simulink model "grid_inv_test_battery"  (R2023a)
settings: Solver=FixedStepDiscrete  StartTime=0.0  StopTime=0.6  FixedStep=5e-6  RelTol=1e-3
libraries: spsSeriesRLCBranchLib x8, slpidlib x4, spsVoltageMeasurementLib x4, spsDiodeLib x3, spsCurrentMeasurementLib x2, spsUniversalBridgeLib x2, spsPVArrayLib x2, spsPWMGenerator2LevelLib x2, spsabctodq0Lib x2, spsDCVoltageSourceLib x1, spsThreePhaseFaultLib x1, spsIGBTLib x1
settings Model: Creator=Umer  LastModifiedBy=Umer

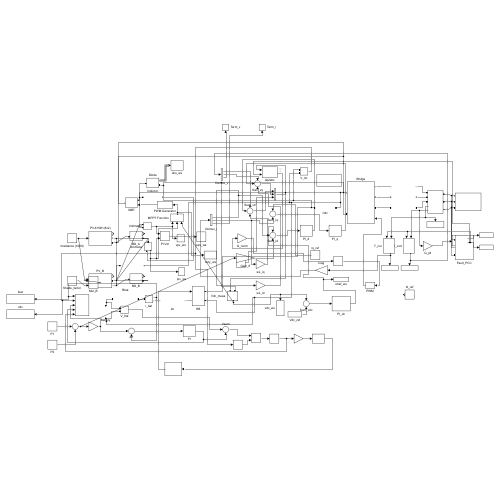
[thumbnail: Simulink's stored preview of the top-level diagram]
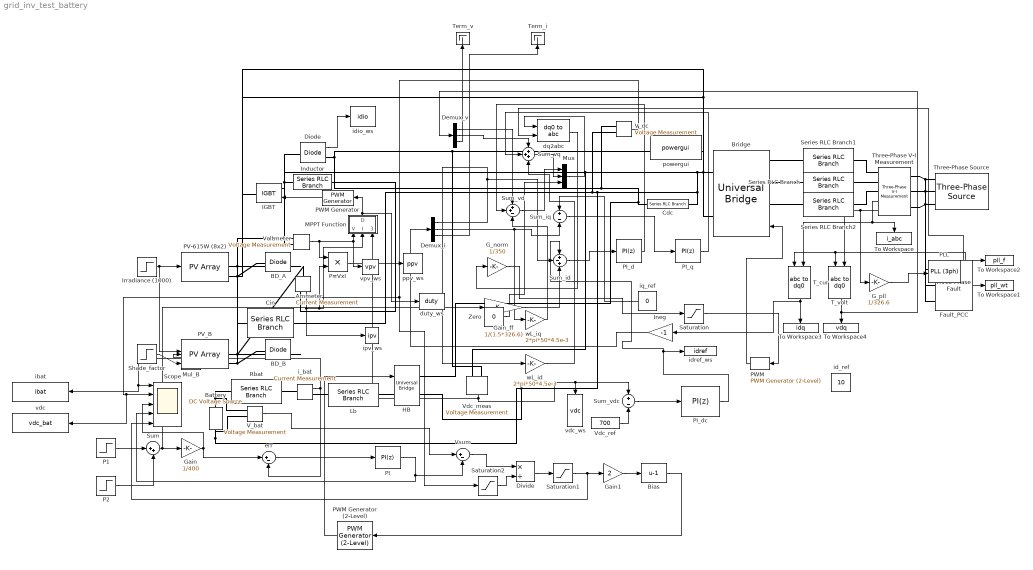
== system grid_inv_test_battery ==
  Ammeter : spsCurrentMeasurementLib/Current Measurement  PhasorSimulation=off  OutputType=Complex  PSBequivalent=0
  BD_A : spsDiodeLib/Diode  Ron=0.001  Lon=0  Vf=0.8  IC=0  UseSnubber=0  Rs=500  Cs=250e-9  Measurements=on
  BD_B : spsDiodeLib/Diode  Ron=0.001  Lon=0  Vf=0.8  IC=0  UseSnubber=0  Rs=500  Cs=250e-9  Measurements=on
  Battery : spsDCVoltageSourceLib/DC Voltage Source  Amplitude=400  Measurements=None
  Bias : Bias  Bias=-1  SaturateOnIntegerOverflow=off
  Bridge : spsUniversalBridgeLib/Universal Bridge  Arms=3  SnubberResistance=1e5  SnubberCapacitance=inf  Device=IGBT / Diodes  Ron=1e-3  Lon=0  ForwardVoltages="[  0  0  ]"  ForwardVoltage=0  GTOparameters=[ 10e-6 , 20e-6 ]  IGBTparameters=[ 1e-6 , 2e-6 ]  Measurements=None  Measurements_2=None  converterType=Rectifier
  Cdc : spsSeriesRLCBranchLib/Series RLC Branch  LConnTagsString=__new0  RConnTagsString=__new0  BranchType=C  Resistance=1  Inductance=1e-3  SetiL0=off  InitialCurrent=0  Capacitance=2e-3  Setx0=on  InitialVoltage=700  Measurements=None
  Cin : spsSeriesRLCBranchLib/Series RLC Branch  LConnTagsString=__new0  RConnTagsString=__new0  BranchType=RC  Resistance=8  Inductance=1e-3  SetiL0=off  InitialCurrent=0  Capacitance=100e-6  Setx0=on  InitialVoltage=380  Measurements=None
  Demux_i : Demux  Outputs=3
  Demux_v : Demux  Outputs=3
  Diode : spsDiodeLib/Diode  Ron=0.001  Lon=0  Vf=0.8  IC=0  UseSnubber=0  Rs=500  Cs=250e-9  Measurements=on
  Divide : Product  Inputs=*/
  Fault_PCC : spsThreePhaseFaultLib/Three-Phase Fault  InitialStates=0  FaultA=on  FaultB=on  FaultC=on  GroundFault=off  SwitchTimes=[10 11]  External=off  SwitchStatus=NaN  FaultResistance=0.001  GroundResistance=0.01  SnubberResistance=1e6  SnubberCapacitance=inf  Measurements=None
  G_norm : Gain  Gain=1/350
  G_pll : Gain  Gain=1/326.6
  Gain : Gain  Gain=1/400
  Gain1 : Gain  Gain=2
  Gain_ff : Gain  Gain=1/(1.5*326.6)
  HB : spsUniversalBridgeLib/Universal Bridge  Arms=1  SnubberResistance=1e5  SnubberCapacitance=inf  Device=IGBT / Diodes  Ron=1e-3  Lon=0  ForwardVoltages="[  0  0  ]"  ForwardVoltage=0  GTOparameters=[ 10e-6 , 20e-6 ]  IGBTparameters=[ 1e-6 , 2e-6 ]  Measurements=None  Measurements_2=None  converterType=Rectifier
  IGBT : spsIGBTLib/IGBT  Ron=0.001  Lon=0  Vf=1  Tf=1e-6  Tt=2e-6  IC=0  Rs=1e5  Cs=1e-6  Measurements=off
  Inductor : spsSeriesRLCBranchLib/Series RLC Branch  LConnTagsString=__new0  RConnTagsString=__new0  BranchType=L  Resistance=0.02  Inductance=7e-3  SetiL0=off  InitialCurrent=0  Capacitance=1e-6  Setx0=off  InitialVoltage=0  Measurements=None
  Ineg : Gain  Gain=-1
  Irradiance (1000) : Step  Time=0.25  Before=300  After=300  SampleTime=0
  Lb : spsSeriesRLCBranchLib/Series RLC Branch  LConnTagsString=__new0  RConnTagsString=__new0  BranchType=RL  Resistance=0.02  Inductance=10e-3  SetiL0=off  InitialCurrent=0  Capacitance=1e-6  Setx0=off  InitialVoltage=0  Measurements=None
  MPPT Function : MATLAB Function  TreatAsAtomicUnit=on
  Mul_B : Product
  Mux : Mux  Inputs=3
  P1 : Step  Time=0.4  After=5000  SampleTime=0
  P2 : Step  Time=0.8  After=-10000  SampleTime=0
  P=VxI : Product
  PI : slpidlib/PID Controller  Controller=PI  Form=Parallel  TimeDomain=Discrete-time  UseExternalTs=off  SampleTime=5e-5  IntegratorMethod=Forward Euler  FilterMethod=Forward Euler  ControllerParametersSource=internal  P=19  I=3600  UseKiTs=off  D=0  N=100  UseFilter=on  TunerSelectOption=Transfer Function Based (PID Tuner App)  InitialConditionSource=internal  InitialConditionForIntegrator=0  InitialConditionForFilter=0  DifferentiatorICPrevScaledInput=0  ExternalReset=none  TrackingMode=off  Kt=1  LimitOutput=off  SatLimitsSource=internal  UpperSaturationLimit=inf  LowerSaturationLimit=-inf  LinearizeAsGain=on  AntiWindupMode=none  Kb=1  LimitIntegrator=off  UpperIntegratorSaturationLimit=inf  LowerIntegratorSaturationLimit=-inf  POutMin=[]  POutMax=[]  IOutMin=[]  IOutMax=[]  DOutMin=[]  DOutMax=[]  NOutMin=[]  NOutMax=[]  SumOutMin=[]  SumOutMax=[]  SaturationOutMin=[]  SaturationOutMax=[]  PParamMin=[]  PParamMax=[]  IParamMin=[]  IParamMax=[]  DParamMin=[]  DParamMax=[]  NParamMin=[]  NParamMax=[]  KbParamMin=[]  KbParamMax=[]  KtParamMin=[]  KtParamMax=[]  KbOutMin=[]  KbOutMax=[]  KtOutMin=[]  KtOutMax=[]  IntegratorOutMin=[]  IntegratorOutMax=[]  FilterOutMin=[]  FilterOutMax=[]  SumI1OutMin=[]  SumI1OutMax=[]  SumI2OutMin=[]  SumI2OutMax=[]  SumI3OutMin=[]  SumI3OutMax=[]  SumI4OutMin=[]  SumI4OutMax=[]  SumDOutMin=[]  SumDOutMax=[]  DifferentiatorOutMin=[]  DifferentiatorOutMax=[]  FilterDiffOutCoefMin=[]  FilterDiffOutCoefMax=[]  ReciprocalOutMin=[]  ReciprocalOutMax=[]  SumDenOutMin=[]  SumDenOutMax=[]  SumNumOutMin=[]  SumNumOutMax=[]  DivideOutMin=[]  DivideOutMax=[]  UdiffTsProdOutMin=[]  UdiffTsProdOutMax=[]  NTsProdOutMin=[]  NTsProdOutMax=[]  UintegralTsProdOutMin=[]  UintegralTsProdOutMax=[]  UngainTsProdOutMin=[]  UngainTsProdOutMax=[]  ClampingZeroOutDataTypeStr=Inherit: Inherit via back propagation  ClampingZeroOutMin=[]  ClampingZeroOutMax=[]  FilterDenConstantOutDataTypeStr=Inherit: Inherit via back propagation  FilterDenConstantOutMin=[]  FilterDenConstantOutMax=[]  PCopyOutDataTypeStr=Inherit: Inherit via back propagation  PCopyOutMin=[]  PCopyOutMax=[]  NCopyOutDataTypeStr=Inherit: Inherit via back propagation  NCopyOutMin=[]  NCopyOutMax=[]  IntegratorContinuousStateAttributes=''  IntegratorStateMustResolveToSignalObject=off  IntegratorRTWStateStorageClass=Auto  FilterContinuousStateAttributes=''  FilterStateMustResolveToSignalObject=off  FilterRTWStateStorageClass=Auto  ParallelPVariant=InternalParameters  IdealPVariant=Disabled  IVariant=InternalParameters  DVariant=Disabled  IntegratorVariant=Discrete  SatVariant=Disabled  AWVariant=Passthrough  PCopyVariant=Disabled  TRVariant=Disabled  FdbkBlocksVariant=Forward  IdealPFdbkVariant=Disabled  SatFdbkVariant=Disabled  DerivativeFilterVariant=Disabled  NVariant=Disabled  NCopyVariant=Disabled_SignalSpec  FilterICVariant=Disabled  IntegratorICVariant=InternalICs  ExternalResetVariant=Disabled  TRSumVariant=Passthrough  SumFdbkVariant=Disabled  SumVariant=Sum_PI  TsampFilterVariant=InternalTs  TsampNgainVariant=Passthrough  TsampIntegralVariant=Disabled_SignalSpec  ExternalSaturationOutDataTypeStr=Inherit: Same as second input
  PI_d : slpidlib/PID Controller  Controller=PI  Form=Parallel  TimeDomain=Discrete-time  UseExternalTs=off  SampleTime=5e-6  IntegratorMethod=Forward Euler  FilterMethod=Forward Euler  ControllerParametersSource=internal  P=10  I=111  UseKiTs=off  D=0  N=100  UseFilter=on  TunerSelectOption=Transfer Function Based (PID Tuner App)  InitialConditionSource=internal  InitialConditionForIntegrator=0  InitialConditionForFilter=0  DifferentiatorICPrevScaledInput=0  ExternalReset=none  TrackingMode=off  Kt=1  LimitOutput=on  SatLimitsSource=internal  UpperSaturationLimit=+350  LowerSaturationLimit=-350  LinearizeAsGain=on  AntiWindupMode=clamping  Kb=1  LimitIntegrator=off  UpperIntegratorSaturationLimit=inf  LowerIntegratorSaturationLimit=-inf  POutMin=[]  POutMax=[]  IOutMin=[]  IOutMax=[]  DOutMin=[]  DOutMax=[]  NOutMin=[]  NOutMax=[]  SumOutMin=[]  SumOutMax=[]  SaturationOutMin=[]  SaturationOutMax=[]  PParamMin=[]  PParamMax=[]  IParamMin=[]  IParamMax=[]  DParamMin=[]  DParamMax=[]  NParamMin=[]  NParamMax=[]  KbParamMin=[]  KbParamMax=[]  KtParamMin=[]  KtParamMax=[]  KbOutMin=[]  KbOutMax=[]  KtOutMin=[]  KtOutMax=[]  IntegratorOutMin=[]  IntegratorOutMax=[]  FilterOutMin=[]  FilterOutMax=[]  SumI1OutMin=[]  SumI1OutMax=[]  SumI2OutMin=[]  SumI2OutMax=[]  SumI3OutMin=[]  SumI3OutMax=[]  SumI4OutMin=[]  SumI4OutMax=[]  SumDOutMin=[]  SumDOutMax=[]  DifferentiatorOutMin=[]  DifferentiatorOutMax=[]  FilterDiffOutCoefMin=[]  FilterDiffOutCoefMax=[]  ReciprocalOutMin=[]  ReciprocalOutMax=[]  SumDenOutMin=[]  SumDenOutMax=[]  SumNumOutMin=[]  SumNumOutMax=[]  DivideOutMin=[]  DivideOutMax=[]  UdiffTsProdOutMin=[]  UdiffTsProdOutMax=[]  NTsProdOutMin=[]  NTsProdOutMax=[]  UintegralTsProdOutMin=[]  UintegralTsProdOutMax=[]  UngainTsProdOutMin=[]  UngainTsProdOutMax=[]  ClampingZeroOutDataTypeStr=Inherit: Inherit via back propagation  ClampingZeroOutMin=[]  ClampingZeroOutMax=[]  FilterDenConstantOutDataTypeStr=Inherit: Inherit via back propagation  FilterDenConstantOutMin=[]  FilterDenConstantOutMax=[]  PCopyOutDataTypeStr=Inherit: Inherit via back propagation  PCopyOutMin=[]  PCopyOutMax=[]  NCopyOutDataTypeStr=Inherit: Inherit via back propagation  NCopyOutMin=[]  NCopyOutMax=[]  IntegratorContinuousStateAttributes=''  IntegratorStateMustResolveToSignalObject=off  IntegratorRTWStateStorageClass=Auto  FilterContinuousStateAttributes=''  FilterStateMustResolveToSignalObject=off  FilterRTWStateStorageClass=Auto  ParallelPVariant=InternalParameters  IdealPVariant=Disabled  IVariant=InternalParameters  DVariant=Disabled  IntegratorVariant=Discrete  SatVariant=Enabled  AWVariant=DiscClampingParallel  PCopyVariant=Disabled  TRVariant=Disabled  FdbkBlocksVariant=Forward  IdealPFdbkVariant=Disabled  SatFdbkVariant=Disabled  DerivativeFilterVariant=Disabled  NVariant=Disabled  NCopyVariant=Disabled_SignalSpec  FilterICVariant=Disabled  IntegratorICVariant=InternalICs  ExternalResetVariant=Disabled  TRSumVariant=Passthrough  SumFdbkVariant=Disabled  SumVariant=Sum_PI  TsampFilterVariant=InternalTs  TsampNgainVariant=Passthrough  TsampIntegralVariant=Disabled_SignalSpec  ExternalSaturationOutDataTypeStr=Inherit: Same as second input
  PI_dc : slpidlib/PID Controller  Controller=PI  Form=Parallel  TimeDomain=Discrete-time  UseExternalTs=off  SampleTime=1e-4  IntegratorMethod=Forward Euler  FilterMethod=Forward Euler  ControllerParametersSource=internal  P=0.3  I=10  UseKiTs=off  D=0  N=100  UseFilter=on  TunerSelectOption=Transfer Function Based (PID Tuner App)  InitialConditionSource=internal  InitialConditionForIntegrator=10  InitialConditionForFilter=0  DifferentiatorICPrevScaledInput=0  ExternalReset=none  TrackingMode=off  Kt=1  LimitOutput=on  SatLimitsSource=internal  UpperSaturationLimit=20  LowerSaturationLimit=-20  LinearizeAsGain=on  AntiWindupMode=clamping  Kb=1  LimitIntegrator=off  UpperIntegratorSaturationLimit=inf  LowerIntegratorSaturationLimit=-inf  POutMin=[]  POutMax=[]  IOutMin=[]  IOutMax=[]  DOutMin=[]  DOutMax=[]  NOutMin=[]  NOutMax=[]  SumOutMin=[]  SumOutMax=[]  SaturationOutMin=[]  SaturationOutMax=[]  PParamMin=[]  PParamMax=[]  IParamMin=[]  IParamMax=[]  DParamMin=[]  DParamMax=[]  NParamMin=[]  NParamMax=[]  KbParamMin=[]  KbParamMax=[]  KtParamMin=[]  KtParamMax=[]  KbOutMin=[]  KbOutMax=[]  KtOutMin=[]  KtOutMax=[]  IntegratorOutMin=[]  IntegratorOutMax=[]  FilterOutMin=[]  FilterOutMax=[]  SumI1OutMin=[]  SumI1OutMax=[]  SumI2OutMin=[]  SumI2OutMax=[]  SumI3OutMin=[]  SumI3OutMax=[]  SumI4OutMin=[]  SumI4OutMax=[]  SumDOutMin=[]  SumDOutMax=[]  DifferentiatorOutMin=[]  DifferentiatorOutMax=[]  FilterDiffOutCoefMin=[]  FilterDiffOutCoefMax=[]  ReciprocalOutMin=[]  ReciprocalOutMax=[]  SumDenOutMin=[]  SumDenOutMax=[]  SumNumOutMin=[]  SumNumOutMax=[]  DivideOutMin=[]  DivideOutMax=[]  UdiffTsProdOutMin=[]  UdiffTsProdOutMax=[]  NTsProdOutMin=[]  NTsProdOutMax=[]  UintegralTsProdOutMin=[]  UintegralTsProdOutMax=[]  UngainTsProdOutMin=[]  UngainTsProdOutMax=[]  ClampingZeroOutDataTypeStr=Inherit: Inherit via back propagation  ClampingZeroOutMin=[]  ClampingZeroOutMax=[]  FilterDenConstantOutDataTypeStr=Inherit: Inherit via back propagation  FilterDenConstantOutMin=[]  FilterDenConstantOutMax=[]  PCopyOutDataTypeStr=Inherit: Inherit via back propagation  PCopyOutMin=[]  PCopyOutMax=[]  NCopyOutDataTypeStr=Inherit: Inherit via back propagation  NCopyOutMin=[]  NCopyOutMax=[]  IntegratorContinuousStateAttributes=''  IntegratorStateMustResolveToSignalObject=off  IntegratorRTWStateStorageClass=Auto  FilterContinuousStateAttributes=''  FilterStateMustResolveToSignalObject=off  FilterRTWStateStorageClass=Auto  ParallelPVariant=InternalParameters  IdealPVariant=Disabled  IVariant=InternalParameters  DVariant=Disabled  IntegratorVariant=Discrete  SatVariant=Enabled  AWVariant=DiscClampingParallel  PCopyVariant=Disabled  TRVariant=Disabled  FdbkBlocksVariant=Forward  IdealPFdbkVariant=Disabled  SatFdbkVariant=Disabled  DerivativeFilterVariant=Disabled  NVariant=Disabled  NCopyVariant=Disabled_SignalSpec  FilterICVariant=Disabled  IntegratorICVariant=InternalICs  ExternalResetVariant=Disabled  TRSumVariant=Passthrough  SumFdbkVariant=Disabled  SumVariant=Sum_PI  TsampFilterVariant=InternalTs  TsampNgainVariant=Passthrough  TsampIntegralVariant=Disabled_SignalSpec  ExternalSaturationOutDataTypeStr=Inherit: Same as second input
  PI_q : slpidlib/PID Controller  Controller=PI  Form=Parallel  TimeDomain=Discrete-time  UseExternalTs=off  SampleTime=5e-6  IntegratorMethod=Forward Euler  FilterMethod=Forward Euler  ControllerParametersSource=internal  P=10  I=111  UseKiTs=off  D=0  N=100  UseFilter=on  TunerSelectOption=Transfer Function Based (PID Tuner App)  InitialConditionSource=internal  InitialConditionForIntegrator=0  InitialConditionForFilter=0  DifferentiatorICPrevScaledInput=0  ExternalReset=none  TrackingMode=off  Kt=1  LimitOutput=on  SatLimitsSource=internal  UpperSaturationLimit=+350  LowerSaturationLimit=-350  LinearizeAsGain=on  AntiWindupMode=clamping  Kb=1  LimitIntegrator=off  UpperIntegratorSaturationLimit=inf  LowerIntegratorSaturationLimit=-inf  POutMin=[]  POutMax=[]  IOutMin=[]  IOutMax=[]  DOutMin=[]  DOutMax=[]  NOutMin=[]  NOutMax=[]  SumOutMin=[]  SumOutMax=[]  SaturationOutMin=[]  SaturationOutMax=[]  PParamMin=[]  PParamMax=[]  IParamMin=[]  IParamMax=[]  DParamMin=[]  DParamMax=[]  NParamMin=[]  NParamMax=[]  KbParamMin=[]  KbParamMax=[]  KtParamMin=[]  KtParamMax=[]  KbOutMin=[]  KbOutMax=[]  KtOutMin=[]  KtOutMax=[]  IntegratorOutMin=[]  IntegratorOutMax=[]  FilterOutMin=[]  FilterOutMax=[]  SumI1OutMin=[]  SumI1OutMax=[]  SumI2OutMin=[]  SumI2OutMax=[]  SumI3OutMin=[]  SumI3OutMax=[]  SumI4OutMin=[]  SumI4OutMax=[]  SumDOutMin=[]  SumDOutMax=[]  DifferentiatorOutMin=[]  DifferentiatorOutMax=[]  FilterDiffOutCoefMin=[]  FilterDiffOutCoefMax=[]  ReciprocalOutMin=[]  ReciprocalOutMax=[]  SumDenOutMin=[]  SumDenOutMax=[]  SumNumOutMin=[]  SumNumOutMax=[]  DivideOutMin=[]  DivideOutMax=[]  UdiffTsProdOutMin=[]  UdiffTsProdOutMax=[]  NTsProdOutMin=[]  NTsProdOutMax=[]  UintegralTsProdOutMin=[]  UintegralTsProdOutMax=[]  UngainTsProdOutMin=[]  UngainTsProdOutMax=[]  ClampingZeroOutDataTypeStr=Inherit: Inherit via back propagation  ClampingZeroOutMin=[]  ClampingZeroOutMax=[]  FilterDenConstantOutDataTypeStr=Inherit: Inherit via back propagation  FilterDenConstantOutMin=[]  FilterDenConstantOutMax=[]  PCopyOutDataTypeStr=Inherit: Inherit via back propagation  PCopyOutMin=[]  PCopyOutMax=[]  NCopyOutDataTypeStr=Inherit: Inherit via back propagation  NCopyOutMin=[]  NCopyOutMax=[]  IntegratorContinuousStateAttributes=''  IntegratorStateMustResolveToSignalObject=off  IntegratorRTWStateStorageClass=Auto  FilterContinuousStateAttributes=''  FilterStateMustResolveToSignalObject=off  FilterRTWStateStorageClass=Auto  ParallelPVariant=InternalParameters  IdealPVariant=Disabled  IVariant=InternalParameters  DVariant=Disabled  IntegratorVariant=Discrete  SatVariant=Enabled  AWVariant=DiscClampingParallel  PCopyVariant=Disabled  TRVariant=Disabled  FdbkBlocksVariant=Forward  IdealPFdbkVariant=Disabled  SatFdbkVariant=Disabled  DerivativeFilterVariant=Disabled  NVariant=Disabled  NCopyVariant=Disabled_SignalSpec  FilterICVariant=Disabled  IntegratorICVariant=InternalICs  ExternalResetVariant=Disabled  TRSumVariant=Passthrough  SumFdbkVariant=Disabled  SumVariant=Sum_PI  TsampFilterVariant=InternalTs  TsampNgainVariant=Passthrough  TsampIntegralVariant=Disabled_SignalSpec  ExternalSaturationOutDataTypeStr=Inherit: Same as second input
  PLL : spsPLL3phLib/PLL (3ph)  Fmin=45  Par_Init=[0, 50]  ParK=[180, 3200, 1]  TcD=1e-4  MaxRateChangeFreq=12  FilterCutOffFreq=25  Ts=50e-6  AGC=on
  PV-615W (8x2) : spsPVArrayLib/PV Array  Npar=2  Nser=4  PlotType=array @ 1000 W/m2 & specified temperatures  S_vec="[ 1000  500  100 ]"  Temp_C_vec="[ 45 25  ]"  ModuleName=User-defined  PlotWhenSelected=off  Pm=615.0834  Ncell=156  Voc=56.25  Isc=13.8  Vm=46.81  Im=13.14  beta_Voc_pc=-0.25  alpha_Isc_pc=0.045  beta_Voc=-0.14062  alpha_Isc=0.00621  IL=13.8306  I0=4.8519e-12  nI=0.48952  Rsh=482.6219  Rs=0.24814  RobustModel=on  RobustCellTemperature=25  BAL=on  Tc=1e-7  Tfilter=1e-7
  PV_B : spsPVArrayLib/PV Array  Npar=2  Nser=4  PlotType=array @ 1000 W/m2 & specified temperatures  S_vec="[ 1000  500  100 ]"  Temp_C_vec="[ 45 25  ]"  ModuleName=User-defined  PlotWhenSelected=off  Pm=615.0834  Ncell=156  Voc=56.25  Isc=13.8  Vm=46.81  Im=13.14  beta_Voc_pc=-0.25  alpha_Isc_pc=0.045  beta_Voc=-0.14062  alpha_Isc=0.00621  IL=13.8306  I0=4.8519e-12  nI=0.48952  Rsh=482.6219  Rs=0.24814  RobustModel=on  RobustCellTemperature=25  BAL=on  Tc=1e-7  Tfilter=1e-7
  PWM : spsPWMGenerator2LevelLib/PWM Generator (2-Level)  ModulatorType=Three-phase bridge (6 pulses)  ModulatorMode=Unsynchronized  Fc=5000  Pc=0  nF=27  MinMax="[ -1  1 ]"  SamplingTechnique=Natural  ModulatingSignals=off  m=0.95  Freq=50  Phase=0  Ts=0  ShowCarrierOutport=off
  PWM Generator : eePwmGenerator/PWM Generator  CarrCount=Up  Tper=0.0002  Tdelay=0  Ts=5e-6
  PWM Generator (2-Level) : spsPWMGenerator2LevelLib/PWM Generator (2-Level)  ModulatorType=Single-phase half-bridge (2 pulses)  ModulatorMode=Unsynchronized  Fc=5000  Pc=90  nF=27  MinMax="[ -1  1 ]"  SamplingTechnique=Natural  ModulatingSignals=off  m=0.8  Freq=60  Phase=0  Ts=5e-6  ShowCarrierOutport=off
  Rbat : spsSeriesRLCBranchLib/Series RLC Branch  LConnTagsString=__new0  RConnTagsString=__new0  BranchType=R  Resistance=0.1  Inductance=1e-3  SetiL0=off  InitialCurrent=0  Capacitance=1e-6  Setx0=off  InitialVoltage=0  Measurements=None
  Saturation : Saturate  UpperLimit=1  LowerLimit=-1
  Saturation1 : Saturate  UpperLimit=0.95  LowerLimit=0.05
  Saturation2 : Saturate
  Scope : Scope  NumInputPorts=5
  Series RLC Branch : spsSeriesRLCBranchLib/Series RLC Branch  LConnTagsString=__new0  RConnTagsString=__new0  BranchType=RL  Resistance=0.05  Inductance=4.5e-3  SetiL0=off  InitialCurrent=0  Capacitance=1e-6  Setx0=off  InitialVoltage=0  Measurements=None
  Series RLC Branch1 : spsSeriesRLCBranchLib/Series RLC Branch  LConnTagsString=__new0  RConnTagsString=__new0  BranchType=RL  Resistance=0.05  Inductance=4.5e-3  SetiL0=off  InitialCurrent=0  Capacitance=1e-6  Setx0=off  InitialVoltage=0  Measurements=None
  Series RLC Branch2 : spsSeriesRLCBranchLib/Series RLC Branch  LConnTagsString=__new0  RConnTagsString=__new0  BranchType=RL  Resistance=0.05  Inductance=4.5e-3  SetiL0=off  InitialCurrent=0  Capacitance=1e-6  Setx0=off  InitialVoltage=0  Measurements=None
  Shade_factor : Step  Time=0.1  Before=1  SampleTime=0
  Sum : Sum  Inputs=|++
  Sum_id : Sum  Inputs=+-+
  Sum_iq : Sum  Inputs=+-
  Sum_vd : Sum  Inputs=++-
  Sum_vdc : Sum  Inputs=+-
  Sum_vq : Sum  Inputs=+++
  T_cur : spsabctodq0Lib/abc to dq0  Alignment=90 degrees behind phase A axis
  T_volt : spsabctodq0Lib/abc to dq0  Alignment=90 degrees behind phase A axis
  Term_i : Terminator
  Term_v : Terminator
  Three-Phase Source : spsThreePhaseSourceLib/Three-Phase Source  InternalConnection=Yg  VoltagePhases=off  Voltage=400  PhaseAngle=0  Voltage_phases=[25e3 25e3 25e3]/sqrt(3)  PhaseAngles_phases=[0 -120 +120]  Frequency=50  NonIdealSource=on  SpecifyImpedance=off  Resistance=0.01  Inductance=1e-4  ShortCircuitLevel=100e6  BaseVoltage=400  XRratio=7  BusType=swing  Pref=10e3  Qref=0  Prefabc=[10e3, 10e3, 10e3]  Qrefabc=[0, 0, 0]  Qmin=-inf  Qmax=inf
  Three-Phase V-I Measurement : spsThreePhaseVIMeasurementLib/Three-Phase V-I Measurement  VoltageMeasurement=phase-to-ground  SetLabelV=off  LabelV=Vabc  Vpu=off  VpuLL=off  CurrentMeasurement=yes  SetLabelI=off  LabelI=Iabc  Ipu=off  Pbase=100e6  Vbase=500e3  OutputType=Complex  PhasorSimulation=off  PSBequivalent=0
  To Workspace : ToWorkspace  VariableName=i_abc  SaveFormat=Timeseries  SampleTime=-1
  To Workspace1 : ToWorkspace  VariableName=pll_wt  SaveFormat=Timeseries  SampleTime=-1
  To Workspace2 : ToWorkspace  VariableName=pll_f  SaveFormat=Timeseries  SampleTime=-1
  To Workspace3 : ToWorkspace  VariableName=idq  SaveFormat=Timeseries  SampleTime=-1
  To Workspace4 : ToWorkspace  VariableName=vdq  SaveFormat=Timeseries  SampleTime=-1
  V_bat : spsVoltageMeasurementLib/Voltage Measurement  PhasorSimulation=off  OutputType=Complex  PSBequivalent=0
  V_dc : spsVoltageMeasurementLib/Voltage Measurement  PhasorSimulation=off  OutputType=Complex  PSBequivalent=0
  Vdc_meas : spsVoltageMeasurementLib/Voltage Measurement  PhasorSimulation=off  OutputType=Complex  PSBequivalent=0
  Vdc_ref : Constant  Value=700
  Voltmeter : spsVoltageMeasurementLib/Voltage Measurement  PhasorSimulation=off  OutputType=Complex  PSBequivalent=0
  Vsum : Sum  Inputs=|+-
  Zero : Constant  Value=0
  dq2abc : spsdq0toabcLib/dq0 to abc  Alignment=90 degrees behind phase A axis
  duty_ws : ToWorkspace  VariableName=duty  SaveFormat=Structure With Time  SampleTime=5e-6
  err : Sum  Inputs=|+-
  i_bat : spsCurrentMeasurementLib/Current Measurement  PhasorSimulation=off  OutputType=Complex  PSBequivalent=0
  ibat : ToWorkspace  VariableName=ibat  SaveFormat=Structure With Time  SampleTime=-1
  id_ref : Constant  Value=10
  idio_ws : ToWorkspace  VariableName=idio  SaveFormat=Structure With Time  SampleTime=5e-6
  idref_ws : ToWorkspace  VariableName=idref  SampleTime=-1
  ipv_ws : ToWorkspace  VariableName=ipv  SaveFormat=Structure With Time  SampleTime=5e-6
  iq_ref : Constant  Value=0
  powergui : spspowerguiLib/powergui  Priority=1  SimulationMode=Discrete  SampleTime=5e-6  frequency=60  Iterations=50  frequencyindice=50  Pbase=100e6  ErrMax=1e-4  UnitsV=kV  UnitsW=MW  buscounter=0  FunctionMessages=off  echomessages=off  EnableUseOfTLC=off  CurrentSourceSwitches=off  DisableSnubberDevices=off  DisableRonSwitches=off  DisableVfSwitches=off  DisplayEquations=off  AutomaticDiscreteSolvers=off  SolverType=Tustin/Backward Euler (TBE)  Interpol=off  ExternalGateDelay=off  methode=off  Ts=100  x0status=blocks  SPID=on  SwTol=0  HookPort=off  NonlinearTolerance=1e-4  nMaxIteration=100  ContinueOnMaxIteration=off  RestoreLinks=warning  ResistiveCurrentMeasurement=off  Frange=[0:2:500]  Ylog=off  Xlog=on  ShowGrid=off  save=off  variable=ZData  structure=0  ZoomFFT=off  StartTime=0.0  cycles=1  DisplayStyle=1  fundamental=60  FreqAxis=off  MaxFrequency=1000  frequencyindicesteady=1  RmsSteady=1  display=off
  ppv_ws : ToWorkspace  VariableName=ppv  SaveFormat=Structure With Time  SampleTime=5e-6
  vdc : ToWorkspace  VariableName=vdc_bat  SaveFormat=Structure With Time  SampleTime=-1
  vdc_ws : ToWorkspace  VariableName=vdc  SampleTime=5e-6
  vpv_ws : ToWorkspace  VariableName=vpv  SaveFormat=Structure With Time  SampleTime=5e-6
  wL_id : Gain  Gain=2*pi*50*4.5e-3
  wL_iq : Gain  Gain=2*pi*50*4.5e-3
  wires:
  G_pll/1 -> PLL/1
  PLL/1 -> To Workspace2/1
  PLL/2 -> To Workspace1/1, T_volt/2, T_cur/2, dq2abc/2
  Three-Phase V-I Measurement/1 -> T_volt/1, G_pll/1
  Three-Phase V-I Measurement/2 -> T_cur/1, To Workspace/1
  T_cur/1 -> To Workspace3/1, Ineg/1
  T_volt/1 -> To Workspace4/1, Demux_v/1
  Demux_i/1 -> Sum_id/2, wL_id/1
  iq_ref/1 -> Sum_iq/1
  Demux_i/2 -> Sum_iq/2, wL_iq/1
  Sum_id/1 -> PI_d/1
  Sum_iq/1 -> PI_q/1
  Demux_v/1 -> Sum_vd/1
  PI_d/1 -> Sum_vd/2
  wL_iq/1 -> Sum_vd/3
  Demux_v/2 -> Sum_vq/1
  PI_q/1 -> Sum_vq/2
  wL_id/1 -> Sum_vq/3
  Sum_vd/1 -> Mux/1
  Sum_vq/1 -> Mux/2
  Zero/1 -> Mux/3
  Mux/1 -> dq2abc/1
  dq2abc/1 -> G_norm/1
  G_norm/1 -> Saturation/1
  Saturation/1 -> PWM/1
  PWM/1 -> Bridge/1
  Demux_i/3 -> Term_i/1
  Demux_v/3 -> Term_v/1
  Ineg/1 -> Demux_i/1
  Vdc_meas/1 -> vdc_ws/1, Sum_vdc/1, MPPT Function/3(Vdc)
  Vdc_ref/1 -> Sum_vdc/2
  Sum_vdc/1 -> PI_dc/1
  PI_dc/1 -> Sum_id/1, idref_ws/1
  Voltmeter/1 -> vpv_ws/1, MPPT Function/1(V), P=VxI/1
  Ammeter/1 -> MPPT Function/2(I), P=VxI/2, ipv_ws/1
  MPPT Function/1(D) -> PWM Generator/1, duty_ws/1
  PWM Generator/1 -> IGBT/1
  P=VxI/1 -> ppv_ws/1
  Diode/1 -> idio_ws/1
  V_dc/1 -> Saturation2/1, vdc/1, Scope/2
  i_bat/1 -> ibat/1, Scope/1, err/2
  P1/1 -> Sum/1
  P2/1 -> Sum/2
  Gain/1 -> err/1, Scope/3
  err/1 -> PI/1
  PI/1 -> Vsum/2, Scope/4
  V_bat/1 -> Vsum/1
  Vsum/1 -> Divide/1
  Divide/1 -> Saturation1/1
  Saturation1/1 -> Gain1/1, Scope/5
  Gain1/1 -> Bias/1
  Bias/1 -> PWM Generator (2-Level)/1
  PWM Generator (2-Level)/1 -> HB/1
  Saturation2/1 -> Divide/2
  Gain_ff/1 -> Sum_id/3
  Irradiance (1000)/1 -> PV-615W (8x2)/1, Mul_B/1
  Shade_factor/1 -> Mul_B/2
  Mul_B/1 -> PV_B/1
  Sum/1 -> Gain/1, Gain_ff/1
  connections:
  Series RLC Branch2/LConn1 -- Bridge/LConn1
  Series RLC Branch1/RConn1 -- Three-Phase V-I Measurement/RConn3
  Series RLC Branch/RConn1 -- Three-Phase V-I Measurement/RConn2
  Series RLC Branch2/RConn1 -- Three-Phase V-I Measurement/RConn1
  Series RLC Branch1/LConn1 -- Bridge/LConn3
  Bridge/LConn2 -- Series RLC Branch/LConn1
  Ammeter/RConn1 -- Inductor/LConn1
  Diode/LConn1 -- Inductor/RConn1 -- IGBT/LConn1
  Bridge/RConn1 -- Diode/RConn1 -- HB/RConn1 -- Cdc/LConn1 -- V_dc/LConn1 -- Vdc_meas/LConn1
  IGBT/RConn1 -- Cin/RConn1 -- V_dc/LConn2 -- V_bat/LConn2 -- Battery/LConn1 -- HB/RConn2 -- Cdc/RConn1 -- Voltmeter/LConn2 -- Vdc_meas/LConn2 -- Bridge/RConn2 -- PV-615W (8x2)/RConn2 -- BD_A/LConn1
  Battery/RConn1 -- Rbat/LConn1 -- V_bat/LConn1
  Rbat/RConn1 -- i_bat/LConn1
  i_bat/RConn1 -- Lb/LConn1
  Lb/RConn1 -- HB/LConn1
  Three-Phase V-I Measurement/LConn1 -- Three-Phase Source/RConn1 -- Fault_PCC/LConn1
  Three-Phase V-I Measurement/LConn2 -- Three-Phase Source/RConn2 -- Fault_PCC/LConn2
  Three-Phase V-I Measurement/LConn3 -- Three-Phase Source/RConn3 -- Fault_PCC/LConn3
  PV-615W (8x2)/RConn1 -- BD_A/RConn1 -- PV_B/RConn2 -- BD_B/LConn1
  Ammeter/LConn1 -- PV_B/RConn1 -- Voltmeter/LConn1 -- Cin/LConn1 -- BD_B/RConn1

== matlab function grid_inv_test_battery/MPPT Function ==
  data: V input; D output; I input; Vdc input
function D = mppt1(V, I, Vdc)
persistent Dprev Pprev Vprev sV sI n
if isempty(Dprev)
    Dprev = 0.5; Pprev = 0; Vprev = 0; sV = 0; sI = 0; n = 0;
end
dD = 0.003; Nn = 2000; Vhi = 735; kv = 0.01;
if Vdc > Vhi
    D = max(0.05, Dprev - kv*(Vdc - Vhi)); sV = 0; sI = 0; n = 0; Pprev = V*I; Vprev = V;
    return
end
sV = sV + V; sI = sI + I; n = n + 1;
if n >= Nn
    Vm = sV/n; Im = sI/n; P = Vm*Im;
    if (P - Pprev) ~= 0
        if (P - Pprev) > 0
            if (Vm - Vprev) > 0, Dprev = Dprev - dD; else, Dprev = Dprev + dD; end
        else
            if (Vm - Vprev) > 0, Dprev = Dprev + dD; else, Dprev = Dprev - dD; end
        end
    end
    if Dprev >= 0.9, Dprev = 0.9; elseif Dprev <= 0.1, Dprev = 0.1; end
    Pprev = P; Vprev = Vm; sV = 0; sI = 0; n = 0;
end
D = Dprev;
end
